simulink library "casper_library_pfbs"  (Simulink 7.2)
settings: Solver=ode45  SolverMode=SingleTasking  StartTime=0.0  StopTime=10.0  RelTol=1e-3
undefined symbols (not defined in the file or in its folder): pfb_coeff_gen_calc
libraries: xbsIndex_r4 x138, casper_library_pfbs x18, casper_library_misc x7, casper_library_delays x7, casper_library_flow_control x2
(part 1 of 3)
settings Model: Creator=mdexter  LastModifiedBy=davidm

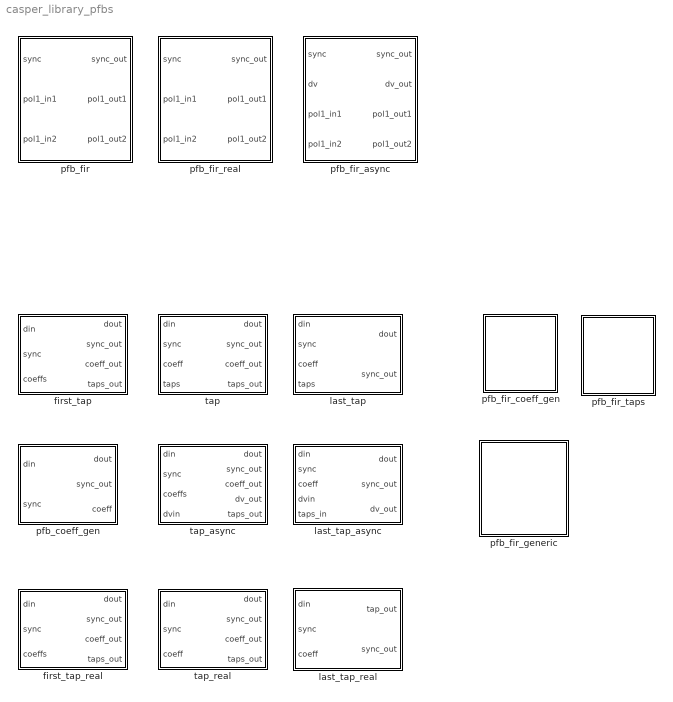
== system casper_library_pfbs ==
  first_tap : Subsystem  mask(first_tap){PFBSize=6, CoeffBitWidth=8, TotalTaps=4, BitWidthIn=8, WindowType=hamming, mult_latency=1, bram_latency=1, n_inputs=2, fwidth=1, use_hdl=off, use_embedded=on}
      mask prompts: PFBSize "Size of PFB: (2^? pnts)"; CoeffBitWidth "Bitwidth of Coefficients:"; TotalTaps "Total Number of Taps:"; BitWidthIn "Input Bitwidth:"; WindowType "Windowing Function:"; mult_latency "Mult Latency"; bram_latency "BRAM Latency"; n_inputs "Number of Simultaneous Inputs: (2^?)"; fwidth "Bit Width (normal=1)"; use_hdl "Use behavioral HDL for multlipliers"; use_embedded "Use embedded multipliers"
      mask init:
      | first_tap_init(gcb,...
      |     'PFBSize', PFBSize,...
      |     'CoeffBitWidth', CoeffBitWidth,...
      |     'TotalTaps', TotalTaps,...
      |     'BitWidthIn', BitWidthIn,...
      |     'WindowType', WindowType,...
      |     'mult_latency', mult_latency,...
      |     'bram_latency', bram_latency,...
      |     'n_inputs', n_inputs,...
      |     'fwidth', fwidth,...
      |     'use_hdl', use_hdl,...
      |     'use_embedded', use_embedded);
      settings: AttributesFormatString=taps=4
      mask StyleString: edit,edit,edit,edit,popup(bartlett|barthannwin|blackman|blackmanharris|bohamwin|chebwin|flattopwin|gausswin|hamming|hann|kaiser|nuttallwin|parzenwin|rectwin|tukeywin|triang),edit,edit,edit,edit,checkbox,checkbox
      mask CallbackString:
      | |||||||||use_hdl = get_param(gcb,'use_hdl');
      | if( strcmp(use_hdl,'on')),
      |     set_param(gcb, 'use_embedded','off');
      |     set_param(gcb, 'MaskVisibilities',{'on','on','on','on','on','on','on','on','on','on','off'});
      | else,
      |     set_param(gcb, 'MaskVisibilities',{'on','on','on','on','on','on','on','on','on','on','on'});
      | end
      | |
  first_tap_real : Subsystem  mask(first_tap_real){PFBSize=6, CoeffBitWidth=8, TotalTaps=4, BitWidthIn=8, WindowType=hamming, mult_latency=1, bram_latency=3, n_inputs=2, fwidth=1, use_hdl=off, use_embedded=on}
      mask prompts: PFBSize "Size of PFB: (2^? pnts)"; CoeffBitWidth "Bitwidth of Coefficients:"; TotalTaps "Total Number of Taps:"; BitWidthIn "Input Bitwidth:"; WindowType "Windowing Function:"; mult_latency "Mult Latency"; bram_latency "BRAM Latency"; n_inputs "Number of Simultaneous Inputs: (2^?)"; fwidth "Bit Width (normal=1)"; use_hdl "Use behavioral HDL for multlipliers"; use_embedded "Use embedded multipliers"
      mask init:
      | first_tap_real_init(gcb,...
      |     'PFBSize', PFBSize,...
      |     'CoeffBitWidth', CoeffBitWidth,...
      |     'TotalTaps', TotalTaps,...
      |     'BitWidthIn', BitWidthIn,...
      |     'WindowType', WindowType,...
      |     'mult_latency', mult_latency,...
      |     'bram_latency', bram_latency,...
      |     'n_inputs', n_inputs,...
      |     'fwidth', fwidth,...
      |     'use_hdl', use_hdl,...
      |     'use_embedded', use_embedded);
      settings: AttributesFormatString=taps=4
      mask StyleString: edit,edit,edit,edit,popup(bartlett|barthannwin|blackman|blackmanharris|bohamwin|chebwin|flattopwin|gausswin|hamming|hann|kaiser|nuttallwin|parzenwin|rectwin|tukeywin|triang|userwindow),edit,edit,edit,edit,checkbox,checkbox
      mask CallbackString:
      | |||||||||use_hdl = get_param(gcb,'use_hdl');
      | if( strcmp(use_hdl,'on')),
      |     set_param(gcb, 'use_embedded','off');
      |     set_param(gcb, 'MaskVisibilities',{'on','on','on','on','on','on','on','on','on','on','off'});
      | else,
      |     set_param(gcb, 'MaskVisibilities',{'on','on','on','on','on','on','on','on','on','on','on'});
      | end
      | |
  last_tap : Subsystem  mask(last_tap){TotalTaps=4, BitWidthIn=8, BitWidthOut=18, CoeffBitWidth=8, add_latency=1, mult_latency=2, quantization=Truncate, use_hdl=off, use_embedded=on}
      mask prompts: TotalTaps "Total Number of Taps:"; BitWidthIn "Input Bitwidth:"; BitWidthOut "Output Bitwidth:"; CoeffBitWidth "Coeff Bitwidth:"; add_latency "Add Latency"; mult_latency "Mult Latency"; quantization "Quantization Behavior"; use_hdl "Use behavioral HDL for multlipliers"; use_embedded "Use embedded multipliers"
      mask init:
      | last_tap_init(gcb,...
      |     'TotalTaps', TotalTaps,...
      |     'BitWidthIn', BitWidthIn,...
      |     'BitWidthOut', BitWidthOut,...
      |     'CoeffBitWidth', CoeffBitWidth,...
      |     'add_latency', add_latency,...
      |     'mult_latency', mult_latency,...
      |     'quantization', quantization,...
      |     'use_hdl', use_hdl,...
      |     'use_embedded', use_embedded);
      settings: AttributesFormatString=taps=4
      mask StyleString: edit,edit,edit,edit,edit,edit,popup(Truncate|Round  (unbiased: +/- Inf)|Round  (unbiased: Even Values)),checkbox,checkbox
      mask CallbackString:
      | |||||||use_hdl = get_param(gcb,'use_hdl');
      | if( strcmp(use_hdl,'on')),
      |     set_param(gcb, 'use_embedded','off');
      |     set_param(gcb, 'MaskVisibilities',{'on','on','on','on','on','on','on','on','off'});
      | else,
      |     set_param(gcb, 'MaskVisibilities',{'on','on','on','on','on','on','on','on','on'});
      | end
      | |
  last_tap_async : Subsystem  mask(last_tap_async){input_num=1, total_taps=2, data_in_bits=8, data_out_bits=18, coeff_bits=8, add_latency=1, mult_latency=2, quantization=Truncate, use_hdl=on, use_embedded=off, async=on, debug_mode=off}
      mask prompts: input_num "Input number:"; total_taps "Total Number of Taps:"; data_in_bits "Input Bitwidth:"; data_out_bits "Output Bitwidth:"; coeff_bits "Coeff Bitwidth:"; add_latency "Add Latency"; mult_latency "Mult Latency"; quantization "Quantization Behavior"; use_hdl "Use behavioral HDL for multlipliers"; use_embedded "Use embedded multipliers"; async "Make asynchronous?"; debug_mode "Debug mode - coeffs are a [1:pfb_size*taps] ramp."
      mask init:
      | last_tap_async_init(gcb,...
      |     'input_num', input_num, ...
      |     'total_taps', total_taps,...
      |     'data_in_bits', data_in_bits,...
      |     'data_out_bits', data_out_bits,...
      |     'coeff_bits', coeff_bits,...
      |     'add_latency', add_latency,...
      |     'mult_latency', mult_latency,...
      |     'quantization', quantization,...
      |     'use_hdl', use_hdl,...
      |     'use_embedded', use_embedded, ...
      |     'async', async, ...
      |     'debug_mode', debug_mode);
      settings: AttributesFormatString=input(1), tap(2,2)
      mask StyleString: edit,edit,edit,edit,edit,edit,edit,popup(Truncate|Round  (unbiased: +/- Inf)|Round  (unbiased: Even Values)),checkbox,checkbox,checkbox,checkbox
      mask CallbackString:
      | ||||||||use_hdl = get_param(gcb,'use_hdl');
      | if( strcmp(use_hdl,'on')),
      |     set_param(gcb, 'use_embedded','off');
      |     set_param(gcb, 'MaskVisibilities',{'on','on','on','on','on','on','on','on','on','off', 'on', 'on'});
      | else
      |     set_param(gcb, 'MaskVisibilities',{'on','on','on','on','on','on','on','on','on','on', 'on', 'on'});
      | end
      | |||
  last_tap_real : Subsystem  mask(last_tap_real){BitWidthIn=8, CoeffBitWidth=8, mult_latency=2, use_hdl=on, use_embedded=off}
      mask prompts: BitWidthIn "Input Bitwidth:"; CoeffBitWidth "Coeff Bitwidth:"; mult_latency "Mult Latency"; use_hdl "Use behavioral HDL for multlipliers"; use_embedded "Use embedded multipliers"
      mask init:
      | last_tap_real_init(gcb,...
      |     'BitWidthIn', BitWidthIn,...
      |     'CoeffBitWidth', CoeffBitWidth,...
      |     'mult_latency', mult_latency,...
      |     'use_hdl', use_hdl,...
      |     'use_embedded', use_embedded);
      mask CallbackString:
      | |||use_hdl = get_param(gcb,'use_hdl');
      | if( strcmp(use_hdl,'on')),
      |     set_param(gcb, 'use_embedded','off');
      |     set_param(gcb, 'MaskVisibilities',{'on','on','on','on','off'});
      | else,
      |     set_param(gcb, 'MaskVisibilities',{'on','on','on','on','on'});
      | end
      | |
  pfb_coeff_gen : Subsystem  mask(pfb_coeff_gen){PFBSize=2, CoeffBitWidth=8, TotalTaps=4, CoeffDistMem=off, WindowType=hamming, bram_latency=2, n_inputs=0, nput=0, fwidth=1, debug_mode=off, fan_latency=1}
      mask prompts: PFBSize "Size of PFB: (2^? pnts)"; CoeffBitWidth "Bitwidth of Coefficients:"; TotalTaps "Total Number of Taps:"; CoeffDistMem "Implement Coeff Gen in Distributed Memory"; WindowType "Windowing Function:"; bram_latency "BRAM Latency"; n_inputs "Number of Simultaneous Inputs: (2^?)"; nput "This is input number:"; fwidth "Bin Width (normal=1)"; debug_mode "Debug mode - coeffs are a [1:pfb_size*taps] ramp."; fan_latency "Fanout latency"
      mask init:
      | pfb_coeff_gen_init(gcb, ...
      |     'PFBSize', PFBSize, ...
      |     'CoeffBitWidth', CoeffBitWidth, ...
      |     'TotalTaps', TotalTaps, ...
      |     'CoeffDistMem', CoeffDistMem, ...
      |     'WindowType', WindowType, ...
      |     'bram_latency', bram_latency, ...
      |     'n_inputs', n_inputs, ...
      |     'nput', nput, ...
      |     'fwidth', fwidth, ...
      |     'fan_latency', fan_latency, ...
      |     'debug_mode', debug_mode);
      settings: AttributesFormatString=|
      | PFBSize=2, n_inputs=0,
      | taps=4, input=0
  pfb_fir : Subsystem  Tag=casper:pfb_fir  mask(pfb_fir){PFBSize=5, TotalTaps=2, WindowType=hamming, n_inputs=1, MakeBiplex=off, BitWidthIn=8, BitWidthOut=18, CoeffBitWidth=18, CoeffDistMem=off, add_latency=1, mult_latency=2, bram_latency=2, fan_latency=1, quantization=Round  (unbiased: Even Values), fwidth=1, mult_spec=2, coeffs_share=on}
      mask prompts: PFBSize "Size of PFB: (2^? pnts)"; TotalTaps "Total Number of Taps:"; WindowType "Windowing Function:"; n_inputs "Number of Simultaneous Inputs: (2^?)"; MakeBiplex "Make Biplex?"; BitWidthIn "Input Bitwidth:"; BitWidthOut "Output Bitwidth:"; CoeffBitWidth "Coefficient Bitwidth:"; CoeffDistMem "Use Distributed Memory for Coeffs"; add_latency "Add Latency"; mult_latency "Mult Latency"; bram_latency "BRAM Latency"; fan_latency "Fanout Latency"; quantization "Quantization Behavior"; fwidth "Bin Width Scaling (normal=1)"; mult_spec "Multiplier specification (0=core, 1=embedded, 2=behavioural) (left=1st tap, or just one value)"; coeffs_share "Share coefficients between polarisations (use less BRAM)?"
      mask init:
      | pfb_fir_init(gcb, ...
      |     'PFBSize', PFBSize, ...
      |     'TotalTaps', TotalTaps, ...
      |     'WindowType', WindowType, ...
      |     'n_inputs', n_inputs, ...
      |     'MakeBiplex', MakeBiplex, ...
      |     'BitWidthIn', BitWidthIn, ...
      |     'BitWidthOut', BitWidthOut, ...
      |     'CoeffBitWidth', CoeffBitWidth, ...
      |     'CoeffDistMem', CoeffDistMem, ...
      |     'add_latency', add_latency, ...
      |     'mult_latency', mult_latency, ...
      |     'bram_latency', bram_latency, ...
      |     'fan_latency', fan_latency, ...
      |     'quantization', quantization, ...
      |     'fwidth', fwidth, ...
      |     'mult_spec', mult_spec, ...
      |     'coeffs_share', coeffs_share);
      settings: AttributesFormatString=|
      | taps=2, add_latency=1
      | max scale 0.500
      mask Help: eval('xlWeb(''http://casper.berkeley.edu/wiki/Pfb_fir'')')
      mask StyleString: edit,edit,popup(bartlett|barthannwin|blackman|blackmanharris|bohamwin|chebwin|flattopwin|gausswin|hamming|hann|kaiser|nuttallwin|parzenwin|rectwin|tukeywin|triang|userwindow),edit,checkbox,edit,edit,edit,checkbox,edit,edit,edit,edit,popup(Truncate|Round  (unbiased: +/- Inf)|Round  (unbiased: Even Values)),edit,edit,checkbox
      mask CallbackString:
      | |%num_taps = eval(get_param(gcb, 'TotalTaps'));
      | %old_vec = eval(get_param(gcb, 'mult_spec'));
      | 
      | %vec = 2.*ones(1,num_taps);
      | %old_size = length(old_vec);
      | 
      | %if(old_size <= num_taps),
      | %   new_size = old_size;
      | %else,
      | %    new_size = num_taps;
      | %end
      | 
      | %for n = 1:new_size, vec(n) = old_vec(n); end
      | %set_param(gcb, 'mult_spec', mat2str(vec));|||||||||||||%num_taps = eval(get_param(gcb, 'TotalTaps'));
      | %old_vec = eval(get_param(gcb, 'mult_spec'));
      | 
      | %vec = 2.*ones(1,num_taps);
      | %old_size = length(old_vec);
      | 
      | %if(old_size <= num_taps),
      | %    new_size = old_size;
      | %else,
      | %    new_size = num_taps;
      | %end
      | 
      | %for n = 1:new_size, vec(n) = old_vec(n); end
      | %set_param(gcb, 'mult_spec', mat2str(vec));|%num_taps = eval(get_param(gcb, 'TotalTaps'));
      | %old_vec = eval(get_param(gcb, 'mult_spec'));
      | 
      | %vec = 2.*ones(1,num_taps);
      | %old_size = length(old_vec);
      | 
      | %if(old_size <= num_taps),
      | %    new_size = old_size;
      | %else,
      | %    new_size = num_taps;
      | %end
      | 
      | %for n = 1:new_size, vec(n) = old_vec(n); end
      | %set_param(gcb, 'mult_spec', mat2str(vec));|
  pfb_fir_async : Subsystem  Tag=casper:pfb_fir_async  mask(pfb_fir_async){pfb_bits=5, total_taps=2, window_type=hamming, simul_bits=1, make_biplex=off, data_in_bits=8, data_out_bits=18, coeff_bits=8, coeffs_in_distmem=off, add_latency=1, mult_latency=2, bram_latency=3, fan_latency=1, quantization=Truncate, fwidth=1, mult_spec=2, coeffs_share=off, async=on, debug_mode=off}
      mask prompts: pfb_bits "Size of PFB: (2^? pnts)"; total_taps "Total Number of Taps:"; window_type "Windowing Function:"; simul_bits "Number of Simultaneous Inputs: (2^?)"; make_biplex "Make Biplex?"; data_in_bits "Input Bitwidth:"; data_out_bits "Output Bitwidth:"; coeff_bits "Coefficient Bitwidth:"; coeffs_in_distmem "Use distributed memory for coeffs"; add_latency "Add Latency"; mult_latency "Mult Latency"; bram_latency "BRAM Latency"; fan_latency "Fanout latency"; quantization "Quantization Behavior"; fwidth "Bin Width Scaling (normal=1)"; mult_spec "Multiplier specification (0=core, 1=embedded, 2=behavioural) (left=1st tap, or just one value)"; coeffs_share "Share coefficients between polarisations (use less BRAM)?"; async "Make asynchronous"; debug_mode "Debug mode - coeffs are a [1:pfb_size*taps] ramp."
      mask init:
      | pfb_fir_async_init(gcb, ...
      |     'pfb_bits', pfb_bits, ...
      |     'total_taps', total_taps, ...
      |     'window_type', window_type, ...
      |     'simul_bits', simul_bits, ...
      |     'make_biplex', make_biplex, ...
      |     'data_in_bits', data_in_bits, ...
      |     'data_out_bits', data_out_bits, ...
      |     'coeff_bits', coeff_bits, ...
      |     'coeffs_in_distmem', coeffs_in_distmem, ...
      |     'add_latency', add_latency, ...
      |     'mult_latency', mult_latency, ...
      |     'bram_latency', bram_latency, ...
      |     'fan_latency', fan_latency, ...
      |     'quantization', quantization, ...
      |     'fwidth', fwidth, ...
      |     'mult_spec', mult_spec, ...
      |     'coeffs_share', coeffs_share, ...
      |     'async', async, ...
      |     'debug_mode', debug_mode);
      settings: AttributesFormatString=|
      | taps=2, add_latency=1
      | max scale 0.500
      mask Help: eval('xlWeb(''http://casper.berkeley.edu/wiki/Pfb_fir'')')
      mask StyleString: edit,edit,popup(bartlett|barthannwin|blackman|blackmanharris|bohamwin|chebwin|flattopwin|gausswin|hamming|hann|kaiser|nuttallwin|parzenwin|rectwin|tukeywin|triang|userwindow),edit,checkbox,edit,edit,edit,checkbox,edit,edit,edit,edit,popup(Truncate|Round  (unbiased: +/- Inf)|Round  (unbiased: Even Values)),edit,edit,checkbox,checkbox,checkbox
  pfb_fir_coeff_gen : Subsystem  mask(pfb_fir_coeff_gen){pfb_size=5, n_taps=0, n_bits_coeff=12, WindowType=hamming, n_inputs=0, fwidth=1, async=off, bram_latency=2, fan_latency=1, add_latency=1, bram_optimization=Area}
      mask prompts: pfb_size "Size of PFB: (2^? pnts)"; n_taps "Total Number of Taps:"; n_bits_coeff "Bitwidth of Coefficients:"; WindowType "Windowing Function:"; n_inputs "Number of Simultaneous Inputs: (2^?)"; fwidth "Bin Width (normal=1)"; async "Asynchronous operation"; bram_latency "BRAM Latency"; fan_latency "Fanout latency"; add_latency "Add latency"; bram_optimization "BRAM optimization"
      mask init:
      | pfb_fir_coeff_gen_init(gcb, ...
      |     'n_inputs', n_inputs, ...
      |     'pfb_size', pfb_size, ...
      |     'n_taps', n_taps, ...
      |     'n_bits_coeff', n_bits_coeff, ...
      |     'WindowType', WindowType, ...
      |     'fwidth', fwidth, ...
      |     'async', async, ...
      |     'bram_latency', bram_latency, ...
      |     'fan_latency', fan_latency, ...
      |     'add_latency', add_latency, ...
      |     'bram_optimization', bram_optimization);
      mask StyleString: edit,edit,edit,popup(bartlett|barthannwin|blackman|blackmanharris|bohamwin|chebwin|flattopwin|gausswin|hamming|hann|kaiser|nuttallwin|parzenwin|rectwin|tukeywin|triang|userwindow),edit,edit,checkbox,edit,edit,edit,popup(Area|Speed)
      mask TabNameString: basic,basic,basic,basic,basic,basic,basic,latency,latency,latency,implementation
  pfb_fir_generic : Subsystem  Tag=casper:pfb_fir_generic  mask(pfb_fir_generic){n_streams=1, PFBSize=5, TotalTaps=0, WindowType=hamming, n_inputs=0, BitWidthIn=8, BitWidthOut=18, CoeffBitWidth=12, complex=off, async=off, add_latency=1, mult_latency=2, bram_latency=2, fan_latency=1, conv_latency=1, quantization=Round  (unbiased: Even Values), fwidth=1, coeffs_bram_optimization=Area, delays_bram_optimization=Area}
      mask prompts: n_streams "Number input streams?"; PFBSize "Size of PFB: (2^? pnts)"; TotalTaps "Total Number of Taps:"; WindowType "Windowing Function:"; n_inputs "Number of Simultaneous Inputs: (2^?)"; BitWidthIn "Input Bitwidth:"; BitWidthOut "Output Bitwidth:"; CoeffBitWidth "Coefficient Bitwidth:"; complex "Complex data inputs"; async "Asynchronous operation"; add_latency "Add Latency"; mult_latency "Mult Latency"; bram_latency "BRAM Latency"; fan_latency "Fanout Latency"; conv_latency "Convert latency"; quantization "Quantization Behavior"; fwidth "Bin Width Scaling (normal=1)"; coeffs_bram_optimization "Coefficient BRAMs optimization"; delays_bram_optimization "Delay BRAMs optimization"
      mask init:
      | pfb_fir_generic_init(gcb, ...
      |     'n_streams', n_streams, ...
      |     'PFBSize', PFBSize, ...
      |     'TotalTaps', TotalTaps, ...
      |     'WindowType', WindowType, ...
      |     'n_inputs', n_inputs, ...
      |     'complex', complex, ...
      |     'BitWidthIn', BitWidthIn, ...
      |     'BitWidthOut', BitWidthOut, ...
      |     'CoeffBitWidth', CoeffBitWidth, ...
      |     'async', async, ...
      |     'add_latency', add_latency, ...
      |     'mult_latency', mult_latency, ...
      |     'bram_latency', bram_latency, ...
      |     'fan_latency', fan_latency, ...
      |     'conv_latency', conv_latency, ...
      |     'quantization', quantization, ...
      |     'fwidth', fwidth, ...
      |     'coeffs_bram_optimization', coeffs_bram_optimization, ...
      |     'delays_bram_optimization', delays_bram_optimization);
      mask StyleString: edit,edit,edit,popup(bartlett|barthannwin|blackman|blackmanharris|bohamwin|chebwin|flattopwin|gausswin|hamming|hann|kaiser|nuttallwin|parzenwin|rectwin|tukeywin|triang|userwindow),edit,edit,edit,edit,checkbox,checkbox,edit,edit,edit,edit,edit,popup(Truncate|Round  (unbiased: +/- Inf)|Round  (unbiased: Even Values)),edit,popup(Area|Speed),popup(Area|Speed)
      mask CallbackString:
      | ||%num_taps = eval(get_param(gcb, 'TotalTaps'));
      | %old_vec = eval(get_param(gcb, 'mult_spec'));
      | 
      | %vec = 2.*ones(1,num_taps);
      | %old_size = length(old_vec);
      | 
      | %if(old_size <= num_taps),
      | %   new_size = old_size;
      | %else,
      | %    new_size = num_taps;
      | %end
      | 
      | %for n = 1:new_size, vec(n) = old_vec(n); end
      | %set_param(gcb, 'mult_spec', mat2str(vec));||||||||||||||%num_taps = eval(get_param(gcb, 'TotalTaps'));
      | %old_vec = eval(get_param(gcb, 'mult_spec'));
      | 
      | %vec = 2.*ones(1,num_taps);
      | %old_size = length(old_vec);
      | 
      | %if(old_size <= num_taps),
      | %    new_size = old_size;
      | %else,
      | %    new_size = num_taps;
      | %end
      | 
      | %for n = 1:new_size, vec(n) = old_vec(n); end
      | %set_param(gcb, 'mult_spec', mat2str(vec));||
      mask TabNameString: basic,basic,basic,implementation,basic,basic,basic,basic,basic,basic,latency,latency,latency,latency,latency,implementation,implementation,implementation,implementation
  pfb_fir_real : Subsystem  Tag=casper:pfb_fir_real  mask(pfb_fir_real){PFBSize=5, TotalTaps=2, WindowType=hamming, n_inputs=1, MakeBiplex=off, BitWidthIn=8, BitWidthOut=18, CoeffBitWidth=18, CoeffDistMem=off, add_latency=1, mult_latency=2, bram_latency=2, fan_latency=1, conv_latency=1, quantization=Round  (unbiased: Even Values), fwidth=1, mult_spec=2, adder_folding=on, adder_imp=Fabric, coeffs_share=off}
      mask prompts: PFBSize "Size of PFB: (2^? pnts)"; TotalTaps "Total Number of Taps:"; WindowType "Windowing Function:"; n_inputs "Number of Simultaneous Inputs: (2^?)"; MakeBiplex "Make Biplex?"; BitWidthIn "Input Bitwidth:"; BitWidthOut "Output Bitwidth:"; CoeffBitWidth "Coefficient Bitwidth:"; CoeffDistMem "Use Distributed Memory for Coeffs"; add_latency "Add Latency"; mult_latency "Mult Latency"; bram_latency "BRAM Latency"; fan_latency "Fanout latency"; conv_latency "Convert latency"; quantization "Quantization Behavior"; fwidth "Bin Width Scaling (normal=1)"; mult_spec "Multiplier specification (0=core, 1=embedded, 2=behavioural) (left=1st tap, or just one value)"; adder_folding "Fold adders into DSPs"; adder_imp "Adder implementation"; coeffs_share "Share coefficients between polarisations (use less BRAM)?"
      mask help:
      | Fold adders into DSPs: Causes adders to be absorbed into DSP blocks (supported in Virtex5)
      | Adder implementation: Cores using Fabric or DSP48 or behavioral HDL
      mask init:
      | pfb_fir_real_init(gcb, ...
      |     'PFBSize', PFBSize, ...
      |     'TotalTaps', TotalTaps, ...
      |     'WindowType', WindowType, ...
      |     'n_inputs', n_inputs, ...
      |     'MakeBiplex', MakeBiplex, ...
      |     'BitWidthIn', BitWidthIn, ...
      |     'BitWidthOut', BitWidthOut, ...
      |     'CoeffBitWidth', CoeffBitWidth, ...
      |     'CoeffDistMem', CoeffDistMem, ...
      |     'add_latency', add_latency, ...
      |     'mult_latency', mult_latency, ...
      |     'bram_latency', bram_latency, ...
      |     'fan_latency', fan_latency, ...
      |     'conv_latency', conv_latency, ...
      |     'quantization', quantization, ...
      |     'fwidth', fwidth, ...
      |     'mult_spec', mult_spec, ...
      |     'adder_folding', adder_folding, ...
      |     'adder_imp', adder_imp, ...
      |     'coeffs_share', coeffs_share);
      settings: AttributesFormatString=taps=2, add_latency=1
      mask Help: eval('xlWeb(''http://casper.berkeley.edu/wiki/Pfb_fir_real'')')
      mask StyleString: edit,edit,popup(bartlett|barthannwin|blackman|blackmanharris|bohamwin|chebwin|flattopwin|gausswin|hamming|hann|kaiser|nuttallwin|parzenwin|rectwin|tukeywin|triang|userwindow),edit,checkbox,edit,edit,edit,checkbox,edit,edit,edit,edit,edit,popup(Truncate|Round  (unbiased: +/- Inf)|Round  (unbiased: Even Values)),edit,edit,checkbox,popup(Behavioral|Fabric|DSP48),checkbox
      mask CallbackString:
      | |%num_taps = eval(get_param(gcb, 'TotalTaps'));
      | %old_vec = eval(get_param(gcb, 'mult_spec'));=-0l
      | 
      | %vec = 2.*ones(1,num_taps);
      | %old_size = length(old_vec);
      | 
      | %if(old_size <= num_taps),
      | %    new_size = old_size;
      | %else,
      | %    new_size = num_taps;
      | %end
      | 
      | %for n = 1:new_size, vec(n) = old_vec(n); end
      | %set_param(gcb, 'mult_spec', mat2str(vec));||||||||||||||||||
  pfb_fir_taps : Subsystem  mask(pfb_fir_taps){n_streams=1, n_inputs=0, pfb_size=5, n_taps=0, n_bits_data=8, n_bits_coeff=12, bin_pt_coeff=11, complex=off, async=off, mult_latency=2, add_latency=1, bram_latency=1, fan_latency=1, multiplier_implementation=behavioral HDL, bram_optimization=Area}
      mask prompts: n_streams "Number simultaneous streams"; n_inputs "Number simultaneous inputs per stream (2^?)"; pfb_size "PFB size (2^? pnts)"; n_taps "Number of taps"; n_bits_data "Data bit width in"; n_bits_coeff "Coefficient bit width"; bin_pt_coeff "Coefficient binary point"; complex "Complex input data"; async "Asynchronous operation"; mult_latency "Multiplier latency"; add_latency "Adder latency"; bram_latency "BRAM latency"; fan_latency "Fanout latency"; multiplier_implementation "Multiplier implementation"; bram_optimization "BRAM optimization"
      mask init:
      | pfb_fir_taps_init(gcb, ...
      |     'n_streams', n_streams, ...
      |     'n_inputs', n_inputs, ...
      |     'pfb_size', pfb_size, ...
      |     'n_taps', n_taps, ...
      |     'n_bits_data', n_bits_data, ...
      |     'n_bits_coeff', n_bits_coeff, ...
      |     'bin_pt_coeff', bin_pt_coeff, ...
      |     'complex', complex, ...
      |     'async', async, ...
      |     'mult_latency', mult_latency, ...
      |     'add_latency', add_latency, ...
      |     'bram_latency', bram_latency, ...
      |     'fan_latency', fan_latency, ...
      |     'multiplier_implementation', multiplier_implementation, ...
      |     'bram_optimization', bram_optimization);
      mask StyleString: edit,edit,edit,edit,edit,edit,edit,checkbox,checkbox,edit,edit,edit,edit,popup(behavioral HDL|standard core|embedded multiplier core),popup(Area|Speed)
      mask TabNameString: basic,basic,basic,basic,basic,basic,basic,basic,basic,latency,latency,latency,latency,implementation,implementation
  tap : Subsystem  mask(tap){mult_latency=2, coeff_width=12, coeff_frac_width=3, delay=4, data_width=8, bram_latency=1, use_hdl=off, use_embedded=on}
      mask prompts: mult_latency "Multiplier Latency"; coeff_width "Coefficient Bit Width In"; coeff_frac_width "Coefficient Fractional Bits"; delay "Data/Sync Delay"; data_width "Data Bit Width In"; bram_latency "BRAM Latency"; use_hdl "Use behavioral HDL for multlipliers"; use_embedded "Use embedded multipliers"
      mask init:
      | use_hdl = get_param(gcb,'use_hdl');
      | use_embedded = get_param(gcb,'use_embedded');
      | set_param(gcb,'LinkStatus','inactive');
      | 
      | set_param([gcb,'/Mult'],'use_embedded',use_embedded);
      | set_param([gcb,'/Mult'],'use_behavioral_HDL',use_hdl);
      | set_param([gcb,'/Mult1'],'use_embedded',use_embedded);
      | set_param([gcb,'/Mult1'],'use_behavioral_HDL',use_hdl);
      mask CallbackString:
      | ||||||use_hdl = get_param(gcb,'use_hdl');
      | if( strcmp(use_hdl,'on')),
      |     set_param(gcb, 'use_embedded','off');
      |     set_param(gcb, 'MaskVisibilities',{'on','on','on','on','on','on','on','off'});
      | else,
      |     set_param(gcb, 'MaskVisibilities',{'on','on','on','on','on','on','on','on'});
      | end
      | |
  tap_async : Subsystem  mask(tap_async){this_tap=1, pfb_bits=5, coeff_bits=8, total_taps=2, data_in_bits=8, mult_latency=2, bram_latency=3, simul_bits=1, fwidth=1, use_hdl=on, use_embedded=off, async=on, debug_mode=off}
      mask prompts: this_tap "Tap number:"; pfb_bits "Size of PFB: (2^? pnts)"; coeff_bits "Bitwidth of Coefficients:"; total_taps "Total Number of Taps:"; data_in_bits "Input Bitwidth:"; mult_latency "Mult Latency"; bram_latency "BRAM Latency"; simul_bits "Number of Simultaneous Inputs: (2^?)"; fwidth "Bit Width (normal=1)"; use_hdl "Use behavioral HDL for multlipliers"; use_embedded "Use embedded multipliers"; async "Make asynchronous?"; debug_mode "Debug mode - coeffs are a [1:pfb_size*taps] ramp."
      mask init:
      | pfb_async_tap_init(gcb,...
      |     'this_tap', this_tap, ...
      |     'pfb_bits', pfb_bits,...
      |     'coeff_bits', coeff_bits,...
      |     'total_taps', total_taps,...
      |     'data_in_bits', data_in_bits,...
      |     'mult_latency', mult_latency,...
      |     'bram_latency', bram_latency,...
      |     'simul_bits', simul_bits,...
      |     'fwidth', fwidth,...
      |     'use_hdl', use_hdl,...
      |     'use_embedded', use_embedded,...
      |     'async', async, ...
      |     'debug_mode', debug_mode);
      settings: AttributesFormatString=tap(1/2)
      mask CallbackString:
      | |||||||||use_hdl = get_param(gcb,'use_hdl');
      | if( strcmp(use_hdl,'on')),
      |     set_param(gcb, 'use_embedded','off');
      |     set_param(gcb, 'MaskVisibilities',{'on','on','on','on','on','on','on','on','on','on','off','on', 'on'});
      | else,
      |     set_param(gcb, 'MaskVisibilities',{'on','on','on','on','on','on','on','on','on','on','on','on', 'on'});
      | end
      | |||
  tap_real : Subsystem  mask(pfb_tap_real){mult_latency=2, coeff_width=12, coeff_frac_width=3, delay=4, data_width=8, bram_latency=1, use_hdl=on, use_embedded=off}
      mask prompts: mult_latency "Multiplier Latency"; coeff_width "Coefficient Bit Width In"; coeff_frac_width "Coefficient Fractional Bits"; delay "Data/Sync Delay"; data_width "Data Bit Width In"; bram_latency "BRAM Latency"; use_hdl "Use behavioral HDL for multlipliers"; use_embedded "Use embedded multipliers"
      mask init:
      | use_hdl = get_param(gcb,'use_hdl');
      | use_embedded = get_param(gcb,'use_embedded');
      | set_param(gcb,'LinkStatus','inactive');
      | 
      | set_param([gcb,'/Mult'],'use_embedded',use_embedded);
      | set_param([gcb,'/Mult'],'use_behavioral_HDL',use_hdl);

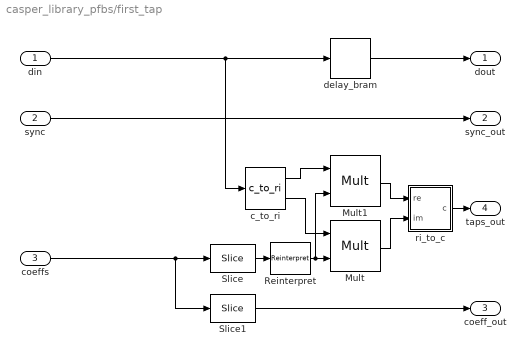
== system casper_library_pfbs/first_tap ==
  din : Inport
  sync : Inport  Port=2
  coeffs : Inport  Port=3
  Mult : xbsIndex_r4/Mult  precision=Full  arith_type="Signed  (2's comp)"  n_bits=8  bin_pt=2  quantization=Truncate  overflow=Wrap  en=off  latency=mult_latency  dbl_ovrd=off  use_behavioral_HDL=off  opt=Speed  use_embedded=on  optimum_pipeline=off  pipeline=on  use_rpm=on  placement_style=Rectangular shape  block_type=mult
      settings: infoedit=Hardware notes: To use the internal pipeline stage of the dedicated multiplier you must select 'Pipeline for maximum performance'.  xl_area=[0, 0, 0, 0, 0, 0, 0]  block_version=9.1.01
  Mult1 : xbsIndex_r4/Mult  precision=Full  arith_type="Signed  (2's comp)"  n_bits=8  bin_pt=2  quantization=Truncate  overflow=Wrap  en=off  latency=mult_latency  dbl_ovrd=off  use_behavioral_HDL=off  opt=Speed  use_embedded=on  optimum_pipeline=off  pipeline=on  use_rpm=on  placement_style=Rectangular shape  block_type=mult
      settings: infoedit=Hardware notes: To use the internal pipeline stage of the dedicated multiplier you must select 'Pipeline for maximum performance'.  xl_area=[0, 0, 0, 0, 0, 0, 0]  block_version=9.1.01
  Reinterpret : xbsIndex_r4/Reinterpret  force_arith_type=on  arith_type="Signed  (2's comp)"  force_bin_pt=on  bin_pt=CoeffBitWidth - 1  block_type=reinterpret
      settings: infoedit="Changes signal type without altering the binary representation.   You can changed the signal between signed and unsigned, and relocate the binary point.<P><P>Hardware notes: In hardware this block costs nothing.<P><P>Example:  Suppose the input is 6 bits wide, signed, with 2 fractional bits, and the output is forced to unsigned with 0 fractional bits.  Then an input of -2.0 (1110.00 in binary 2's complement) becomes an output of 56 (111000 in binary)."  block_version=9.1.01
  Slice : xbsIndex_r4/Slice  nbits=CoeffBitWidth  boolean_output=off  mode=Lower Bit Location + Width  bit1=0  base1=MSB of Input  bit0=0  base0=LSB of Input  dbl_ovrd=off  block_type=slice
      settings: infoedit="Extracts a given range of bits from each input sample and presents it at the output.  The output type is ordinarily unsigned with binary point at zero, but can be Boolean when the slice is one bit wide.<P><P>Hardware notes: In hardware this block costs nothing."  block_version=9.1.01
  Slice1 : xbsIndex_r4/Slice  nbits=CoeffBitWidth * (TotalTaps - 1)  boolean_output=off  mode=Two Bit Locations  bit1=0  base1=MSB of Input  bit0=CoeffBitWidth  base0=LSB of Input  dbl_ovrd=off  block_type=slice
      settings: infoedit="Extracts a given range of bits from each input sample and presents it at the output.  The output type is ordinarily unsigned with binary point at zero, but can be Boolean when the slice is one bit wide.<P><P>Hardware notes: In hardware this block costs nothing."  block_version=9.1.01
  c_to_ri : casper_library_misc/c_to_ri  n_bits=BitWidthIn  bin_pt=BitWidthIn-1
      settings: AttributesFormatString=_ r/i
  delay_bram : casper_library_delays/delay_bram  DelayLen=2^(PFBSize-n_inputs)  bram_latency=bram_latency  use_dsp48=off  async=off
  ri_to_c : Subsystem
  dout : Outport
  sync_out : Outport  Port=2
  coeff_out : Outport  Port=3
  taps_out : Outport  Port=4
  wires:
  Reinterpret/1 -> Mult/2, Mult1/2
  Slice/1 -> Reinterpret/1
  Slice1/1 -> coeff_out/1
  delay_bram/1 -> dout/1
  din/1 -> delay_bram/1, c_to_ri/1
  sync/1 -> sync_out/1
  c_to_ri/1 -> Mult1/1
  c_to_ri/2 -> Mult/1
  Mult1/1 -> ri_to_c/1(re)
  Mult/1 -> ri_to_c/2(im)
  ri_to_c/1(c) -> taps_out/1
  coeffs/1 -> Slice/1, Slice1/1

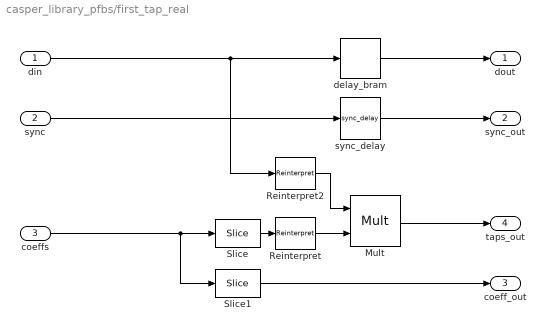
== system casper_library_pfbs/first_tap_real ==
  din : Inport
  sync : Inport  Port=2
  coeffs : Inport  Port=3
  Mult : xbsIndex_r4/Mult  precision=Full  arith_type="Signed  (2's comp)"  n_bits=8  bin_pt=2  quantization=Truncate  overflow=Wrap  en=off  latency=mult_latency  dbl_ovrd=off  use_behavioral_HDL=off  opt=Speed  use_embedded=on  optimum_pipeline=off  pipeline=on  use_rpm=on  placement_style=Rectangular shape  block_type=mult
      settings: infoedit=Hardware notes: To use the internal pipeline stage of the dedicated multiplier you must select 'Pipeline for maximum performance'.  xl_area=[0, 0, 0, 0, 0, 0, 0]  block_version=9.1.01
  Reinterpret : xbsIndex_r4/Reinterpret  force_arith_type=on  arith_type="Signed  (2's comp)"  force_bin_pt=on  bin_pt=CoeffBitWidth - 1  block_type=reinterpret
      settings: infoedit="Changes signal type without altering the binary representation.   You can changed the signal between signed and unsigned, and relocate the binary point.<P><P>Hardware notes: In hardware this block costs nothing.<P><P>Example:  Suppose the input is 6 bits wide, signed, with 2 fractional bits, and the output is forced to unsigned with 0 fractional bits.  Then an input of -2.0 (1110.00 in binary 2's complement) becomes an output of 56 (111000 in binary)."  block_version=9.1.01
  Reinterpret2 : xbsIndex_r4/Reinterpret  force_arith_type=on  arith_type="Signed  (2's comp)"  force_bin_pt=on  bin_pt=BitWidthIn - 1  block_type=reinterpret
      settings: infoedit="Changes signal type without altering the binary representation.   You can changed the signal between signed and unsigned, and relocate the binary point.<P><P>Hardware notes: In hardware this block costs nothing.<P><P>Example:  Suppose the input is 6 bits wide, signed, with 2 fractional bits, and the output is forced to unsigned with 0 fractional bits.  Then an input of -2.0 (1110.00 in binary 2's complement) becomes an output of 56 (111000 in binary)."  block_version=9.1.01
  Slice : xbsIndex_r4/Slice  nbits=CoeffBitWidth  boolean_output=off  mode=Lower Bit Location + Width  bit1=0  base1=MSB of Input  bit0=0  base0=LSB of Input  dbl_ovrd=off  block_type=slice
      settings: infoedit="Extracts a given range of bits from each input sample and presents it at the output.  The output type is ordinarily unsigned with binary point at zero, but can be Boolean when the slice is one bit wide.<P><P>Hardware notes: In hardware this block costs nothing."  block_version=9.1.01
  Slice1 : xbsIndex_r4/Slice  nbits=CoeffBitWidth * (TotalTaps - 1)  boolean_output=off  mode=Two Bit Locations  bit1=0  base1=MSB of Input  bit0=CoeffBitWidth  base0=LSB of Input  dbl_ovrd=off  block_type=slice
      settings: infoedit="Extracts a given range of bits from each input sample and presents it at the output.  The output type is ordinarily unsigned with binary point at zero, but can be Boolean when the slice is one bit wide.<P><P>Hardware notes: In hardware this block costs nothing."  block_version=9.1.01
  delay_bram : casper_library_delays/delay_bram  DelayLen=2^(PFBSize-n_inputs)  bram_latency=bram_latency  use_dsp48=off  async=off
  sync_delay : casper_library_delays/sync_delay  DelayLen=2^(PFBSize-n_inputs)
  dout : Outport
  sync_out : Outport  Port=2
  coeff_out : Outport  Port=3
  taps_out : Outport  Port=4
  wires:
  sync/1 -> sync_delay/1
  din/1 -> delay_bram/1, Reinterpret2/1
  Mult/1 -> taps_out/1
  delay_bram/1 -> dout/1
  sync_delay/1 -> sync_out/1
  Slice1/1 -> coeff_out/1
  Slice/1 -> Reinterpret/1
  Reinterpret/1 -> Mult/2
  Reinterpret2/1 -> Mult/1
  coeffs/1 -> Slice/1, Slice1/1

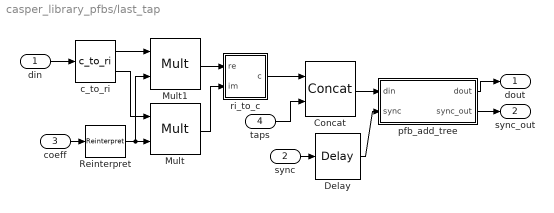
== system casper_library_pfbs/last_tap ==
  din : Inport
  sync : Inport  Port=2
  coeff : Inport  Port=3
  taps : Inport  Port=4
  Concat : xbsIndex_r4/Concat  num_inputs=2  dbl_ovrd=off  block_type=concat
      settings: block_version=9.1.01
  Delay : xbsIndex_r4/Delay  rst=off  infoeditControl=Selection of Reset will increase slice count due to use of real FFs and instead of SRLs  en=off  latency=mult_latency  dbl_ovrd=off  reg_retiming=on  block_type=delay
      settings: xl_area=[0, 0, 0, 0, 0, 0, 0]  block_version=9.1.01
  Mult : xbsIndex_r4/Mult  precision=Full  arith_type="Signed  (2's comp)"  n_bits=8  bin_pt=2  quantization=Truncate  overflow=Wrap  en=off  latency=mult_latency  dbl_ovrd=off  use_behavioral_HDL=off  opt=Speed  use_embedded=on  optimum_pipeline=off  pipeline=on  use_rpm=on  placement_style=Rectangular shape  block_type=mult
      settings: infoedit=Hardware notes: To use the internal pipeline stage of the dedicated multiplier you must select 'Pipeline for maximum performance'.  xl_area=[0, 0, 0, 0, 0, 0, 0]  block_version=9.1.01
  Mult1 : xbsIndex_r4/Mult  precision=Full  arith_type="Signed  (2's comp)"  n_bits=8  bin_pt=2  quantization=Truncate  overflow=Wrap  en=off  latency=mult_latency  dbl_ovrd=off  use_behavioral_HDL=off  opt=Speed  use_embedded=on  optimum_pipeline=off  pipeline=on  use_rpm=on  placement_style=Rectangular shape  block_type=mult
      settings: infoedit=Hardware notes: To use the internal pipeline stage of the dedicated multiplier you must select 'Pipeline for maximum performance'.  xl_area=[0, 0, 0, 0, 0, 0, 0]  block_version=9.1.01
  Reinterpret : xbsIndex_r4/Reinterpret  force_arith_type=on  arith_type="Signed  (2's comp)"  force_bin_pt=on  bin_pt=CoeffBitWidth - 1  block_type=reinterpret
      settings: infoedit="Changes signal type without altering the binary representation.   You can changed the signal between signed and unsigned, and relocate the binary point.<P><P>Hardware notes: In hardware this block costs nothing.<P><P>Example:  Suppose the input is 6 bits wide, signed, with 2 fractional bits, and the output is forced to unsigned with 0 fractional bits.  Then an input of -2.0 (1110.00 in binary 2's complement) becomes an output of 56 (111000 in binary)."  block_version=9.1.01
  c_to_ri : casper_library_misc/c_to_ri  n_bits=BitWidthIn  bin_pt=BitWidthIn-1
      settings: AttributesFormatString=_ r/i
  pfb_add_tree : Subsystem  mask(pfb_add_tree){TotalTaps=4, BitWidthIn=8, BitWidthOut=18, CoeffBitWidth=8, add_latency=1, quantization=Truncate}
      mask prompts: TotalTaps "Total Number of Taps:"; BitWidthIn "Input Bitwidth:"; BitWidthOut "Output Bitwidth:"; CoeffBitWidth "Coeff Bitwidth:"; add_latency "Add Latency"; quantization "Quantization Behavior"
      mask init:
      | pfb_add_tree_init(gcb, ...
      |     'TotalTaps', TotalTaps, ...
      |     'BitWidthIn', BitWidthIn, ...
      |     'BitWidthOut', BitWidthOut, ...
      |     'CoeffBitWidth', CoeffBitWidth, ...
      |     'add_latency', add_latency, ...
      |     'quantization', quantization);
      settings: AttributesFormatString=taps=4, add_latency=1
      mask StyleString: edit,edit,edit,edit,edit,popup(Truncate|Round  (unbiased: +/- Inf)|Round  (unbiased: Even Values))
  ri_to_c : Subsystem
  dout : Outport
  sync_out : Outport  Port=2
  wires:
  ri_to_c/1(c) -> Concat/1
  Mult/1 -> ri_to_c/2(im)
  Mult1/1 -> ri_to_c/1(re)
  din/1 -> c_to_ri/1
  c_to_ri/2 -> Mult/1
  c_to_ri/1 -> Mult1/1
  Delay/1 -> pfb_add_tree/2(sync)
  pfb_add_tree/2(sync_out) -> sync_out/1
  pfb_add_tree/1(dout) -> dout/1
  sync/1 -> Delay/1
  taps/1 -> Concat/2
  Concat/1 -> pfb_add_tree/1(din)
  coeff/1 -> Reinterpret/1
  Reinterpret/1 -> Mult1/2, Mult/2

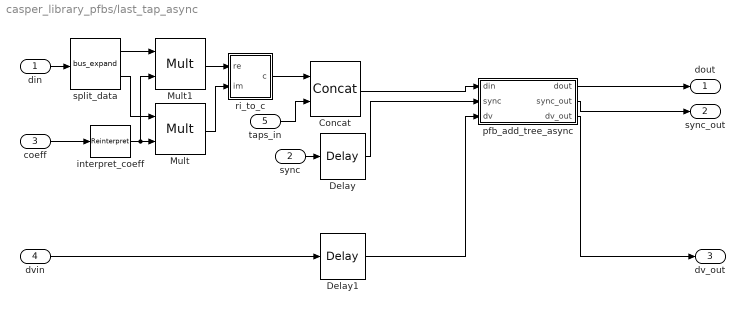
== system casper_library_pfbs/last_tap_async ==
  din : Inport
  sync : Inport  Port=2
  coeff : Inport  Port=3
  dvin : Inport  Port=4
  taps_in : Inport  Port=5
  Concat : xbsIndex_r4/Concat  num_inputs=2  dbl_ovrd=off  block_type=concat
      settings: block_version=9.1.01
  Delay : xbsIndex_r4/Delay  rst=off  infoeditControl=Selection of Reset will increase slice count due to use of real FFs and instead of SRLs  en=off  latency=mult_latency  dbl_ovrd=off  reg_retiming=on  block_type=delay
      settings: xl_area=[0, 0, 0, 0, 0, 0, 0]  block_version=9.1.01
  Delay1 : xbsIndex_r4/Delay  rst=off  infoeditControl=Selection of Reset will increase slice count due to use of real FFs and instead of SRLs  en=off  latency=mult_latency  dbl_ovrd=off  reg_retiming=on  block_type=delay
      settings: xl_area=[0, 0, 0, 0, 0, 0, 0]  block_version=9.1.01
  Mult : xbsIndex_r4/Mult  precision=Full  arith_type="Signed  (2's comp)"  n_bits=8  bin_pt=2  quantization=Truncate  overflow=Wrap  en=off  latency=mult_latency  dbl_ovrd=off  use_behavioral_HDL=on  opt=Speed  use_embedded=off  optimum_pipeline=off  pipeline=on  use_rpm=on  placement_style=Rectangular shape  block_type=mult
      settings: infoedit=Hardware notes: To use the internal pipeline stage of the dedicated multiplier you must select 'Pipeline for maximum performance'.  xl_area=[0, 0, 0, 0, 0, 0, 0]  block_version=9.1.01
  Mult1 : xbsIndex_r4/Mult  precision=Full  arith_type="Signed  (2's comp)"  n_bits=8  bin_pt=2  quantization=Truncate  overflow=Wrap  en=off  latency=mult_latency  dbl_ovrd=off  use_behavioral_HDL=on  opt=Speed  use_embedded=off  optimum_pipeline=off  pipeline=on  use_rpm=on  placement_style=Rectangular shape  block_type=mult
      settings: infoedit=Hardware notes: To use the internal pipeline stage of the dedicated multiplier you must select 'Pipeline for maximum performance'.  xl_area=[0, 0, 0, 0, 0, 0, 0]  block_version=9.1.01
  interpret_coeff : xbsIndex_r4/Reinterpret  force_arith_type=on  arith_type="Signed  (2's comp)"  force_bin_pt=on  bin_pt=coeff_bits - 1  block_type=reinterpret
      settings: infoedit="Changes signal type without altering the binary representation.   You can changed the signal between signed and unsigned, and relocate the binary point.<br><br>Hardware notes: In hardware this block costs nothing.<br><br>Example:  Suppose the input is 6 bits wide, signed, with 2 fractional bits, and the output is forced to unsigned with 0 fractional bits.  Then an input of -2.0 (1110.00 in binary 2's complement) becomes an output of 56 (111000 in binary)."  block_version=9.1.01
  pfb_add_tree_async : Subsystem  mask(pfb_add_tree_async){input_num=1, total_taps=2, data_in_bits=8, data_out_bits=18, coeff_bits=8, add_latency=1, quantization=Truncate, debug_mode=off}
      mask prompts: input_num "Input number:"; total_taps "Total number of taps:"; data_in_bits "Input bitwidth:"; data_out_bits "Output bitwidth:"; coeff_bits "Coeff bitwidth:"; add_latency "Add latency"; quantization "Quantization behavior"; debug_mode "Debug mode - coeffs are a [1:pfb_size*taps] ramp."
      mask init:
      | pfb_add_tree_async_init(gcb, ...
      |     'input_num', input_num, ...
      |     'total_taps', total_taps, ...
      |     'data_in_bits', data_in_bits, ...
      |     'data_out_bits', data_out_bits, ...
      |     'coeff_bits', coeff_bits, ...
      |     'add_latency', add_latency, ...
      |     'quantization', quantization, ...
      |     'debug_mode', debug_mode);
      settings: AttributesFormatString=input(1), taps(2), add_lat(1)
      mask StyleString: edit,edit,edit,edit,edit,edit,popup(Truncate|Round  (unbiased: +/- Inf)|Round  (unbiased: Even Values)),checkbox
  ri_to_c : Subsystem
  split_data : casper_library_flow_control/bus_expand  mode=divisions of equal size  outputNum=2  outputWidth=data_in_bits  outputBinaryPt=data_in_bits - 1  outputArithmeticType=1  show_format=off  outputToWorkspace=off  variablePrefix=out  outputToModelAsWell=on
      settings: AttributesFormatString=2 outputs
  dout : Outport
  sync_out : Outport  Port=2
  dv_out : Outport  Port=3
  wires:
  interpret_coeff/1 -> Mult/2, Mult1/2
  coeff/1 -> interpret_coeff/1
  Concat/1 -> pfb_add_tree_async/1(din)
  taps_in/1 -> Concat/2
  sync/1 -> Delay/1
  pfb_add_tree_async/1(dout) -> dout/1
  pfb_add_tree_async/2(sync_out) -> sync_out/1
  Delay/1 -> pfb_add_tree_async/2(sync)
  split_data/1 -> Mult1/1
  split_data/2 -> Mult/1
  din/1 -> split_data/1
  Mult1/1 -> ri_to_c/1(re)
  Mult/1 -> ri_to_c/2(im)
  ri_to_c/1(c) -> Concat/1
  dvin/1 -> Delay1/1
  pfb_add_tree_async/3(dv_out) -> dv_out/1
  Delay1/1 -> pfb_add_tree_async/3(dv)

== system casper_library_pfbs/last_tap_real ==
  din : Inport
  sync : Inport  Port=2
  coeff : Inport  Port=3
  Delay : xbsIndex_r4/Delay  rst=off  infoeditControl=Selection of Reset will increase slice count due to use of real FFs and instead of SRLs  en=off  latency=mult_latency  dbl_ovrd=off  reg_retiming=on  block_type=delay
      settings: xl_area=[0, 0, 0, 0, 0, 0, 0]  block_version=9.1.01
  Mult : xbsIndex_r4/Mult  precision=Full  arith_type="Signed  (2's comp)"  n_bits=8  bin_pt=2  quantization=Truncate  overflow=Wrap  en=off  latency=mult_latency  dbl_ovrd=off  use_behavioral_HDL=on  opt=Speed  use_embedded=off  optimum_pipeline=off  pipeline=on  use_rpm=on  placement_style=Rectangular shape  block_type=mult
      settings: infoedit=Hardware notes: To use the internal pipeline stage of the dedicated multiplier you must select 'Pipeline for maximum performance'.  xl_area=[0, 0, 0, 0, 0, 0, 0]  block_version=9.1.01
  Reinterpret : xbsIndex_r4/Reinterpret  force_arith_type=on  arith_type="Signed  (2's comp)"  force_bin_pt=on  bin_pt=CoeffBitWidth - 1  block_type=reinterpret
      settings: infoedit="Changes signal type without altering the binary representation.   You can changed the signal between signed and unsigned, and relocate the binary point.<P><P>Hardware notes: In hardware this block costs nothing.<P><P>Example:  Suppose the input is 6 bits wide, signed, with 2 fractional bits, and the output is forced to unsigned with 0 fractional bits.  Then an input of -2.0 (1110.00 in binary 2's complement) becomes an output of 56 (111000 in binary)."  block_version=9.1.01
  Reinterpret1 : xbsIndex_r4/Reinterpret  force_arith_type=on  arith_type="Signed  (2's comp)"  force_bin_pt=on  bin_pt=BitWidthIn - 1  block_type=reinterpret
      settings: infoedit="Changes signal type without altering the binary representation.   You can changed the signal between signed and unsigned, and relocate the binary point.<P><P>Hardware notes: In hardware this block costs nothing.<P><P>Example:  Suppose the input is 6 bits wide, signed, with 2 fractional bits, and the output is forced to unsigned with 0 fractional bits.  Then an input of -2.0 (1110.00 in binary 2's complement) becomes an output of 56 (111000 in binary)."  block_version=9.1.01
  tap_out : Outport
  sync_out : Outport  Port=2
  wires:
  Reinterpret1/1 -> Mult/1
  Mult/1 -> tap_out/1
  Reinterpret/1 -> Mult/2
  coeff/1 -> Reinterpret/1
  sync/1 -> Delay/1
  din/1 -> Reinterpret1/1
  Delay/1 -> sync_out/1
